simulink model "DP_STD_MDL_DCAC_3ph_2level_resload_2022b"  (R2022b)
settings: Solver=VariableStepAuto  StartTime=0.0  StopTime=6  RelTol=1e-3
libraries: spsSeriesRLCBranchLib x18, spsSecondOrderFilterLib x7, spsVoltageMeasurementLib x7, spsMosfetLib x4, simulink x2, spsControlledVoltageSourceLib x1, gmp_sil_core_pack x1, gmp_peripheral_utilities x1, spspowerguiLib x1
(part 1 of 2)
settings Model: SimulationMode=accelerator  Creator=javnson  LastModifiedBy=javnson
settings DataIOCC: ReturnWorkspaceOutputs=off
settings OptimizationCC: ReuseModelBlockBuffer=on
settings RTWCC: GPUComputeCapability=5.0

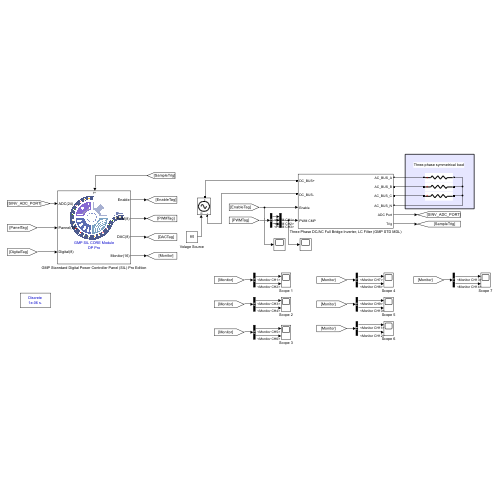
[thumbnail: Simulink's stored preview of the top-level diagram]
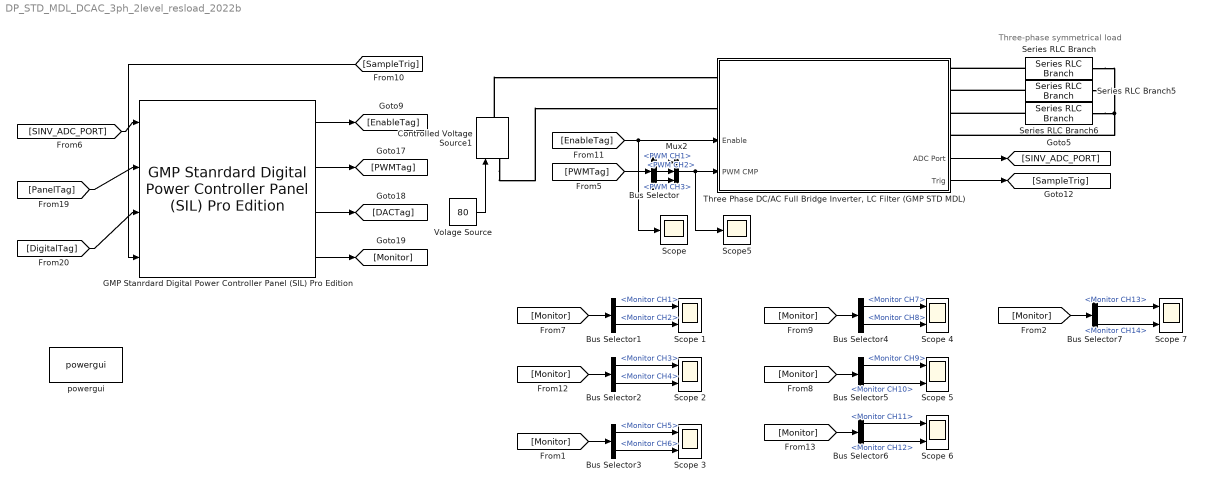
== system DP_STD_MDL_DCAC_3ph_2level_resload_2022b ==
  note: Three-phase symmetrical load
  Bus Selector : BusSelector  OutputSignals=PWM CH1,PWM CH2,PWM CH3
  Bus Selector1 : BusSelector  OutputSignals=Monitor CH1,Monitor CH2
  Bus Selector2 : BusSelector  OutputSignals=Monitor CH3,Monitor CH4
  Bus Selector3 : BusSelector  OutputSignals=Monitor CH5,Monitor CH6
  Bus Selector4 : BusSelector  OutputSignals=Monitor CH7,Monitor CH8
  Bus Selector5 : BusSelector  OutputSignals=Monitor CH9,Monitor CH10
  Bus Selector6 : BusSelector  OutputSignals=Monitor CH11,Monitor CH12
  Bus Selector7 : BusSelector  OutputSignals=Monitor CH13,Monitor CH14
  Controlled Voltage Source1 : spsControlledVoltageSourceLib/Controlled Voltage Source  Initialize=on  Source_Type=AC  Amplitude=0  Phase=0  Frequency=0  Measurements=None
  GMP Stanrdard Digital Power Controller Panel (SIL) Pro Edition : gmp_sil_core_pack/GMP Stanrdard Digital Power Controller Panel (SIL) Pro Edition
      settings: SourceProductName=GMP SIL Core Utilities
  Mux2 : Mux  Inputs=3
  Scope : Scope
  Scope {1..7} (7 alike) : Scope  NumInputPorts=2
  Scope5 : Scope
  Series RLC Branch : spsSeriesRLCBranchLib/Series RLC Branch  LConnTagsString=__new0  RConnTagsString=__new0  BranchType=R  Resistance=50/3  Inductance=1e-3  SetiL0=off  InitialCurrent=0  Capacitance=1e-6  Setx0=off  InitialVoltage=0  Measurements=None
  Series RLC Branch5 : spsSeriesRLCBranchLib/Series RLC Branch  LConnTagsString=__new0  RConnTagsString=__new0  BranchType=R  Resistance=50/3  Inductance=1e-3  SetiL0=off  InitialCurrent=0  Capacitance=1e-6  Setx0=off  InitialVoltage=0  Measurements=None
  Series RLC Branch6 : spsSeriesRLCBranchLib/Series RLC Branch  LConnTagsString=__new0  RConnTagsString=__new0  BranchType=R  Resistance=50/3  Inductance=1e-3  SetiL0=off  InitialCurrent=0  Capacitance=1e-6  Setx0=off  InitialVoltage=0  Measurements=None
  "Three Phase DC/AC Full Bridge Inverter, LC Filter (GMP STD MDL)" : Subsystem  mask{R_mosfet_on=0.001, Lon=0, Rd=0.01, Vf=0.5, Rs=1e5, Cs=inf, ACF_L=1.5e-3, ACF_L_ESR=50e-3, ACF_C=5e-6, ACF_C_ESR=0.09, ACF_C_EPR=10e3, DC_CAP=220e-6*3, DC_CAP_ESR=0.05, DC_CAP_EPR=10e3, fswitch=20e3, CMP_MAX=3000, Deadband_Upper=50, Deadband_Lower=50, phase_shift=0, ADC_Resolution=12, DC_Voltage_Gain=0.02738589, DC_VOLTAGE_ADC_REFERENCE=3.3, DC_VOLTAGE_ADC_BIAS=0, DC_VOLTAGE_ADC_CUT_FREQ=1e3, DC_BUS_CURRENT_SENSOR_R=0.001, DC_Current_Gain=24.75, DC_CURRENT_ADC_REFERENCE=3.3, DC_CURRENT_ADC_BIAS=1.65, DC_CURRENT_ADC_CUT_FREQ=100e3, AC_Voltage_Gain=0.04125, AC_VOLTAGE_ADC_REFERENCE=3.3, AC_VOLTAGE_ADC_BIAS=1.65, AC_VOLTAGE_ADC_CUT_FREQ=1e3, ADC_AC_R_SENSOR=0.001, AC_Current_Gain=48, AC_CURRENT_ADC_REFERENCE=3.3, AC_CURRENT_ADC_BIAS=1.65, AC_CURRENT_ADC_INIT=0, CAP_CURRENT_SENSOR_R=0.001, CAP_Current_Gain=20, CAP_CURRENT_ADC_REFERENCE=3.3, CAP_CURRENT_ADC_BIAS=1.65, CAP_CURRENT_ADC_CUT_FREQ=18e3, GRID_CURRENT_SENSOR_R=0.001, Grid_Current_Gain=48, GRID_CURRENT_ADC_REFERENCE=3.3, GRID_CURRENT_ADC_BIAS=1.65, GRID_CURRENT_ADC_CUT_FREQ=100e3}
      mask prompts: ADC_Resolution "ADC_BIT:"; DC_Voltage_Gain "ADC_GAIN:"; DC_VOLTAGE_ADC_REFERENCE "ADC_REFERENCE:"; DC_VOLTAGE_ADC_BIAS "ADC_BIAS:"; DC_VOLTAGE_ADC_CUT_FREQ "cut_frequency:"; DC_Current_Gain "ADC_GAIN:"; DC_CURRENT_ADC_REFERENCE "ADC_REFERENCE:"; DC_CURRENT_ADC_BIAS "ADC_BIAS:"; DC_CURRENT_ADC_CUT_FREQ "ADC_FILTER:"; AC_Voltage_Gain "ADC_GAIN:"; AC_VOLTAGE_ADC_REFERENCE "ADC_REFERENCE:"; AC_VOLTAGE_ADC_BIAS "ADC_BIAS:"; AC_VOLTAGE_ADC_CUT_FREQ "cut_frequency:"; ADC_AC_R_SENSOR "ADC_DC_R_SENSOR:"; AC_Current_Gain "ADC_GAIN:"; AC_CURRENT_ADC_REFERENCE "ADC_REFERENCE:"; AC_CURRENT_ADC_BIAS "ADC_BIAS:"; AC_CURRENT_ADC_INIT "ADC_INIT:"; CAP_CURRENT_SENSOR_R "CAP_BUS_CURRENT_SENSOR_R:"; CAP_Current_Gain "ADC_GAIN:"; CAP_CURRENT_ADC_REFERENCE "ADC_REFERENCE:"; CAP_CURRENT_ADC_BIAS "ADC_BIAS:"; CAP_CURRENT_ADC_CUT_FREQ "ADC_FILTER:"; GRID_CURRENT_SENSOR_R "DC_BUS_CURRENT_SENSOR_R:"; Grid_Current_Gain "ADC_GAIN:"; GRID_CURRENT_ADC_REFERENCE "ADC_REFERENCE:"; GRID_CURRENT_ADC_BIAS "ADC_BIAS:"; GRID_CURRENT_ADC_CUT_FREQ "ADC_FILTER:"
      settings: PortSchema="{\"entries\":[{\"content\":{\"sides\":[{\"content\":{\"connectorIds\":[\"LConn1\",\"LConn2\",\"In1\",\"In2\"]},\"type\":\"ConnectorPlacement.EquallySpacedRectSide\",\"uuid\":\"0e3e6e75-5e1a-455b-8a22-c69d0a4261ca\"},{\"content\":{\"connectorIds\":[\"RConn1\",\"RConn2\",\"RConn3\",\"RConn4\",\"Out1\",\"Out2\"],\"side\":\"RIGHT\"},\"type\":\"ConnectorPlacement.EquallySpacedRectSide\",\"uuid\":\"20326781-9238-4fea-80fd-ba96906d5d3f\"},{\"content\":{\"side\":\"TOP\"},\"type\":\"ConnectorPlacement.EquallySpacedRectSide\",\"uuid\":\"9e3289d3-0bee-4337-807b-c293a46cda9c\"}]},\"type\":\"ConnectorPlacement.EquallySpacedConnector\",\"uuid\":\"56bb35ad-d602-4874-b9bf-b95a81ef662c\"}],\"packageUris\":[\"http://schema.mathworks.com/mf0/Connector/R2020b\"],\"version\":\"1.0\"}"
      mask DialogControl ParameterGroupVar Prompt: 参数
      mask DialogControl Container4 Prompt: Component Parameters
      mask DialogControl Container7 Prompt: MOSFET
      mask DialogControl Control2 Prompt: Rds(on), unit Ohm
      mask DialogControl Control3 Prompt: Internal diode inducctance, unit H
      mask DialogControl Control4 Prompt: Internal diode resistance Rd, unit Ohm
      mask DialogControl Control5 Prompt: Internal diode forward voltage Vf, unit V
      mask DialogControl Control6 Prompt: Snubber resistance Rs, unit ohm
      mask DialogControl Control7 Prompt: Snubber Capacitance Cs, unit F
      mask DialogControl Container8 Prompt: LC Filter
      mask DialogControl Container20 Prompt: Filter Inductor
      mask DialogControl Control8 Prompt: AC Bus Filter Inductor (H)
      mask DialogControl Control42 Prompt: AC Bus Filter Inductor, ESR (Ohm)
      mask DialogControl Container21 Prompt: Filter Capcitor
      mask DialogControl Control43 Prompt: AC Bus Filter Capacitor (F)
      mask DialogControl Control44 Prompt: AC Bus Filter Capacitor, ESR (Ohm)
      mask DialogControl Control45 Prompt: AC Bus Filter Capacitor, EPR (Ohm)
      mask DialogControl Container22 Prompt: DC Bus Capacitor
      mask DialogControl Control46 Prompt: DC Bus Capacitor (F)
      mask DialogControl Control47 Prompt: DC Bus Capacitor, ESR (Ohm)
      mask DialogControl Control48 Prompt: DC Bus Capacitor, EPR (Ohm)
      mask DialogControl Container5 Prompt: PWM Parameers
      mask DialogControl Control9 Prompt: PWM Frequency (Hz):
      mask DialogControl Control10 Prompt: Full Scale PWM Compare value:
      mask DialogControl Control11 Prompt: (whole period is 2 * CMP_MAX ticks)
      mask DialogControl Control12 Prompt: Deadband Range Set (CMP Value):
      mask DialogControl Control13 Prompt: Single side deadband time: DEADBAND_CMP/2/CMP_MAX/fswitch
      mask DialogControl Control14 Prompt: Initial Phase Shift, unit rad
      mask DialogControl Container6 Prompt: ADC Parameters
      mask DialogControl Container14 Prompt: ADC Device
      mask DialogControl Control15 Prompt: ADC resolution:
      mask DialogControl Container15 Prompt: DC Side Voltage Sensor
      mask DialogControl Control16 Prompt: ADC Voltage Gain (Scale Factor):
      mask DialogControl Control17 Prompt: ADC reference Voltage(V)
      mask DialogControl Control18 Prompt: ADC Bias Voltage(V)
      mask DialogControl Control19 Prompt: Voltage Filter cut frequency (Hz):
      mask DialogControl Control20 Prompt: Generally, this value less than switch frequency / 10, greater than motor normal frequency * 3
      mask DialogControl Container16 Prompt: DC Side Current Sensor
      mask DialogControl Control26 Prompt: DC Bus Current Sensor Resistance
      mask DialogControl Control34 Prompt: ADC Current Gain (Scale Factor):
      mask DialogControl Control27 Prompt: ADC reference Voltage(V), ADC full scale current (when gain = 1)
      mask DialogControl Control28 Prompt: ADC Bias Current(A)
      mask DialogControl Control35 Prompt: Voltage Filter cut frequency (Hz):
      mask DialogControl Control36 Prompt: Generally, this value less than switch frequency / 10, greater than motor normal frequency * 3
      mask DialogControl Container17 Prompt: AC Side Voltage Sensor
      mask DialogControl Control16_copy Prompt: ADC Voltage Gain (Scale Factor):
      mask DialogControl Control17_copy Prompt: ADC reference Voltage(V)
      mask DialogControl Control18_copy Prompt: ADC Bias Voltage(V)
      mask DialogControl Control19_copy Prompt: Voltage Filter cut frequency (Hz):
      mask DialogControl Control20_copy Prompt: Generally, this value less than switch frequency / 10, greater than motor normal frequency * 3
      mask DialogControl Container18 Prompt: AC Side Current Sensor(NC)
      mask DialogControl Control55 Prompt: AC Current Sensor Resistance
      mask DialogControl Control26_copy Prompt: ADC Current Gain (Scale Factor):
      mask DialogControl Control27_copy Prompt: ADC reference Current(A), ADC full scale current (when gain = 1)
      mask DialogControl Control28_copy Prompt: ADC Bias Current(A)
      mask DialogControl Control29_copy Prompt: ADC initial Current Output(A)
      mask DialogControl Container19 Prompt: Capcitor Current Sensor(NC)
      mask DialogControl Control26_copy_copy Prompt: Filter Capacitor Current Sensor Resistance
      mask DialogControl Control34_copy Prompt: ADC Current Gain (Scale Factor):
      mask DialogControl Control27_copy_copy Prompt: ADC reference Voltage(V), ADC full scale current (when gain = 1)
      mask DialogControl Control28_copy_copy Prompt: ADC Bias Current(V)
      mask DialogControl Control35_copy Prompt: Voltage Filter cut frequency (Hz):
      mask DialogControl Control36_copy Prompt: Generally, this value less than switch frequency / 10, greater than motor normal frequency * 3
      mask DialogControl Container23 Prompt: Grid Current Sensor
      mask DialogControl Control26_copy_copy_copy Prompt: Grid Bus Current Sensor Resistance
      mask DialogControl Control34_copy_copy Prompt: ADC Current Gain (Scale Factor):
      mask DialogControl Control27_copy_copy_copy Prompt: ADC reference Voltage(V), ADC full scale current (when gain = 1)
      mask DialogControl Control28_copy_copy_copy Prompt: ADC Bias Current(V)
      mask DialogControl Control35_copy_copy Prompt: Voltage Filter cut frequency (Hz):
      mask DialogControl Control36_copy_copy Prompt: Generally, this value less than switch frequency / 10, greater than motor normal frequency * 3
  Volage Source : Constant  Value=80
  powergui : spspowerguiLib/powergui  Priority=1  SimulationMode=Discrete  SampleTime=1e-6  frequency=60  Iterations=50  frequencyindice=0  Pbase=100e6  ErrMax=1e-4  UnitsV=kV  UnitsW=MW  buscounter=0  FunctionMessages=off  echomessages=off  EnableUseOfTLC=off  CurrentSourceSwitches=off  DisableSnubberDevices=off  DisableRonSwitches=off  DisableVfSwitches=off  DisplayEquations=off  AutomaticDiscreteSolvers=off  SolverType=Tustin/Backward Euler (TBE)  Interpol=off  ExternalGateDelay=off  methode=off  Ts=100  x0status=blocks  SPID=on  SwTol=0  HookPort=off  NonlinearTolerance=1e-4  nMaxIteration=100  ContinueOnMaxIteration=off  RestoreLinks=warning  ResistiveCurrentMeasurement=off  Frange=[0:2:500]  Ylog=off  Xlog=on  ShowGrid=off  save=off  variable=ZData  structure=0  ZoomFFT=off  StartTime=0.0  cycles=1  DisplayStyle=1  fundamental=60  FreqAxis=off  MaxFrequency=1000  frequencyindicesteady=1  RmsSteady=1  display=off
  wires:
  Volage Source/1 -> Controlled Voltage Source1/1
  [EnableTag] -> "Three Phase DC/AC Full Bridge Inverter, LC Filter (GMP STD MDL)"/1(Enable), Scope/1
  [SampleTrig] -> GMP Stanrdard Digital Power Controller Panel (SIL) Pro Edition/4
  GMP Stanrdard Digital Power Controller Panel (SIL) Pro Edition/1 -> [EnableTag]
  GMP Stanrdard Digital Power Controller Panel (SIL) Pro Edition/2 -> [PWMTag]
  GMP Stanrdard Digital Power Controller Panel (SIL) Pro Edition/3 -> [DACTag]
  GMP Stanrdard Digital Power Controller Panel (SIL) Pro Edition/4 -> [Monitor]
  [SINV_ADC_PORT] -> GMP Stanrdard Digital Power Controller Panel (SIL) Pro Edition/1
  [PanelTag] -> GMP Stanrdard Digital Power Controller Panel (SIL) Pro Edition/2
  [DigitalTag] -> GMP Stanrdard Digital Power Controller Panel (SIL) Pro Edition/3
  [PWMTag] -> Bus Selector/1
  Bus Selector/1 -> Mux2/1  "<PWM CH1>"
  Bus Selector/2 -> Mux2/2  "<PWM CH2>"
  Mux2/1 -> "Three Phase DC/AC Full Bridge Inverter, LC Filter (GMP STD MDL)"/2(PWM CMP), Scope5/1
  [Monitor] -> Bus Selector1/1
  Bus Selector1/1 -> Scope 1/1  "<Monitor CH1>"
  Bus Selector1/2 -> Scope 1/2  "<Monitor CH2>"
  [Monitor] -> Bus Selector2/1
  Bus Selector2/1 -> Scope 2/1  "<Monitor CH3>"
  Bus Selector2/2 -> Scope 2/2  "<Monitor CH4>"
  Bus Selector3/2 -> Scope 3/2  "<Monitor CH6>"
  Bus Selector3/1 -> Scope 3/1  "<Monitor CH5>"
  [Monitor] -> Bus Selector3/1
  Bus Selector5/2 -> Scope 5/2  "<Monitor CH10>"
  Bus Selector5/1 -> Scope 5/1  "<Monitor CH9>"
  [Monitor] -> Bus Selector5/1
  [Monitor] -> Bus Selector4/1
  Bus Selector4/1 -> Scope 4/1  "<Monitor CH7>"
  Bus Selector4/2 -> Scope 4/2  "<Monitor CH8>"
  [Monitor] -> Bus Selector6/1
  Bus Selector6/1 -> Scope 6/1  "<Monitor CH11>"
  "Three Phase DC/AC Full Bridge Inverter, LC Filter (GMP STD MDL)"/1(ADC Port) -> [SINV_ADC_PORT]
  "Three Phase DC/AC Full Bridge Inverter, LC Filter (GMP STD MDL)"/2(Trig) -> [SampleTrig]
  Bus Selector/3 -> Mux2/3  "<PWM CH3>"
  Bus Selector6/2 -> Scope 6/2  "<Monitor CH12>"
  Bus Selector7/2 -> Scope 7/2  "<Monitor CH14>"
  Bus Selector7/1 -> Scope 7/1  "<Monitor CH13>"
  [Monitor] -> Bus Selector7/1
  connections:
  Controlled Voltage Source1/LConn1 -- "Three Phase DC/AC Full Bridge Inverter, LC Filter (GMP STD MDL)"/LConn2
  Controlled Voltage Source1/RConn1 -- "Three Phase DC/AC Full Bridge Inverter, LC Filter (GMP STD MDL)"/LConn1
  Series RLC Branch/LConn1 -- "Three Phase DC/AC Full Bridge Inverter, LC Filter (GMP STD MDL)"/RConn1
  Series RLC Branch5/LConn1 -- "Three Phase DC/AC Full Bridge Inverter, LC Filter (GMP STD MDL)"/RConn2
  Series RLC Branch6/LConn1 -- "Three Phase DC/AC Full Bridge Inverter, LC Filter (GMP STD MDL)"/RConn3
  Series RLC Branch/RConn1 -- Series RLC Branch5/RConn1 -- Series RLC Branch6/RConn1 -- "Three Phase DC/AC Full Bridge Inverter, LC Filter (GMP STD MDL)"/RConn4

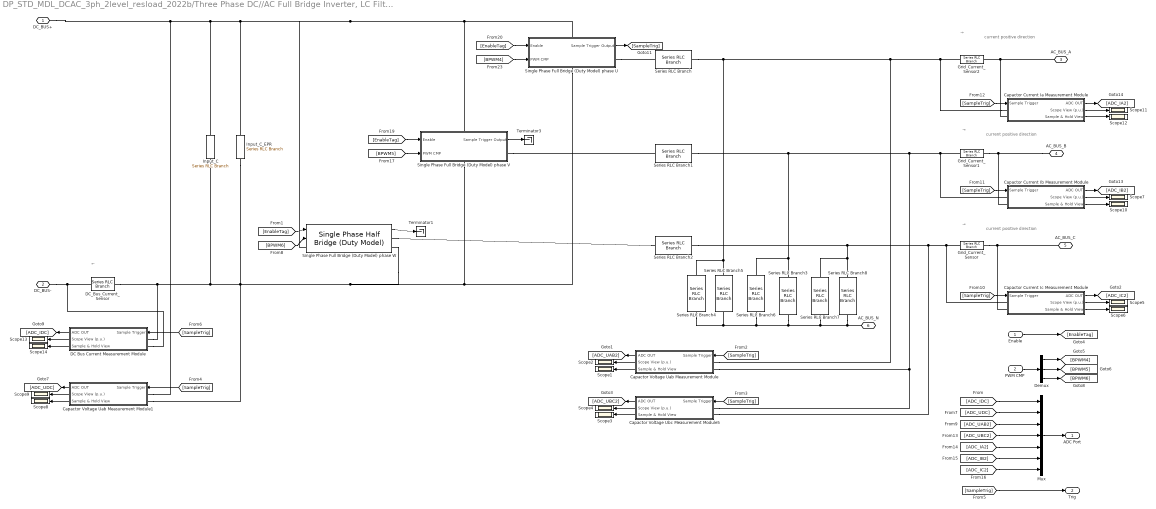
== system DP_STD_MDL_DCAC_3ph_2level_resload_2022b/Three Phase DC//AC Full Bridge Inverter, LC Filter (GMP STD MDL) ==
  note: ←
  note: →
  note: current positive direction
  note: →
  note: current positive direction
  note: →
  note: current positive direction
  Enable : Inport
  PWM CMP : Inport  Port=2
  Capactor Current Ia Measurement Module : Subsystem  mask{ADC_GAIN=Grid_Current_Gain, ADC_BIT=ADC_Resolution, ADC_REFERENCE=GRID_CURRENT_ADC_REFERENCE, ADC_BIAS=GRID_CURRENT_ADC_BIAS, ADC_INIT=0, cut_frequency=GRID_CURRENT_ADC_CUT_FREQ}
      mask DialogControl DescGroupVar Prompt: Voltage Sample ADC Model
      mask DialogControl DescTextVar Prompt: This is a ideal Voltage Measurement Module.
      mask DialogControl Control2 Prompt: ADC(p.u.) = (real_voltage * ADC_GAIN + ADC_BIAS)/ADC_REFERENCE
      mask DialogControl Control11 Prompt: GMP CTL Simulink Utilities: virtual peripherals
      mask DialogControl ParameterGroupVar Prompt: Parameters:
      mask DialogControl Control4 Prompt: ADC Voltage Gain (Scale Factor):
      mask DialogControl Control5 Prompt: ADC resolution:
      mask DialogControl Control6 Prompt: ADC reference Voltage(V)
      mask DialogControl Control8 Prompt: ADC Bias Voltage(V)
      mask DialogControl Control7 Prompt: ADC Initial Voltage Output (V):
      mask DialogControl Control9 Prompt: Voltage Filter cut frequency (Hz):
      mask DialogControl Control10 Prompt: Generally, this value less than switch frequency / 10, greater than motor normal frequency * 3
  Capactor Current Ib Measurement Module : Subsystem  mask{ADC_GAIN=Grid_Current_Gain, ADC_BIT=ADC_Resolution, ADC_REFERENCE=GRID_CURRENT_ADC_REFERENCE, ADC_BIAS=GRID_CURRENT_ADC_BIAS, ADC_INIT=0, cut_frequency=GRID_CURRENT_ADC_CUT_FREQ}
      mask DialogControl DescGroupVar Prompt: Voltage Sample ADC Model
      mask DialogControl DescTextVar Prompt: This is a ideal Voltage Measurement Module.
      mask DialogControl Control2 Prompt: ADC(p.u.) = (real_voltage * ADC_GAIN + ADC_BIAS)/ADC_REFERENCE
      mask DialogControl Control11 Prompt: GMP CTL Simulink Utilities: virtual peripherals
      mask DialogControl ParameterGroupVar Prompt: Parameters:
      mask DialogControl Control4 Prompt: ADC Voltage Gain (Scale Factor):
      mask DialogControl Control5 Prompt: ADC resolution:
      mask DialogControl Control6 Prompt: ADC reference Voltage(V)
      mask DialogControl Control8 Prompt: ADC Bias Voltage(V)
      mask DialogControl Control7 Prompt: ADC Initial Voltage Output (V):
      mask DialogControl Control9 Prompt: Voltage Filter cut frequency (Hz):
      mask DialogControl Control10 Prompt: Generally, this value less than switch frequency / 10, greater than motor normal frequency * 3
  Capactor Current Ic Measurement Module : Subsystem  mask{ADC_GAIN=Grid_Current_Gain, ADC_BIT=ADC_Resolution, ADC_REFERENCE=GRID_CURRENT_ADC_REFERENCE, ADC_BIAS=GRID_CURRENT_ADC_BIAS, ADC_INIT=0, cut_frequency=GRID_CURRENT_ADC_CUT_FREQ}
      mask DialogControl DescGroupVar Prompt: Voltage Sample ADC Model
      mask DialogControl DescTextVar Prompt: This is a ideal Voltage Measurement Module.
      mask DialogControl Control2 Prompt: ADC(p.u.) = (real_voltage * ADC_GAIN + ADC_BIAS)/ADC_REFERENCE
      mask DialogControl Control11 Prompt: GMP CTL Simulink Utilities: virtual peripherals
      mask DialogControl ParameterGroupVar Prompt: Parameters:
      mask DialogControl Control4 Prompt: ADC Voltage Gain (Scale Factor):
      mask DialogControl Control5 Prompt: ADC resolution:
      mask DialogControl Control6 Prompt: ADC reference Voltage(V)
      mask DialogControl Control8 Prompt: ADC Bias Voltage(V)
      mask DialogControl Control7 Prompt: ADC Initial Voltage Output (V):
      mask DialogControl Control9 Prompt: Voltage Filter cut frequency (Hz):
      mask DialogControl Control10 Prompt: Generally, this value less than switch frequency / 10, greater than motor normal frequency * 3
  Capactor Voltage Uab Measurement Module : Subsystem  mask{ADC_GAIN=AC_Voltage_Gain, ADC_BIT=ADC_Resolution, ADC_REFERENCE=AC_VOLTAGE_ADC_REFERENCE, ADC_BIAS=AC_VOLTAGE_ADC_BIAS, ADC_INIT=0, cut_frequency=AC_VOLTAGE_ADC_CUT_FREQ}
      mask DialogControl DescGroupVar Prompt: Voltage Sample ADC Model
      mask DialogControl DescTextVar Prompt: This is a ideal Voltage Measurement Module.
      mask DialogControl Control2 Prompt: ADC(p.u.) = (real_voltage * ADC_GAIN + ADC_BIAS)/ADC_REFERENCE
      mask DialogControl Control11 Prompt: GMP CTL Simulink Utilities: virtual peripherals
      mask DialogControl ParameterGroupVar Prompt: Parameters:
      mask DialogControl Control4 Prompt: ADC Voltage Gain (Scale Factor):
      mask DialogControl Control5 Prompt: ADC resolution:
      mask DialogControl Control6 Prompt: ADC reference Voltage(V)
      mask DialogControl Control8 Prompt: ADC Bias Voltage(V)
      mask DialogControl Control7 Prompt: ADC Initial Voltage Output (V):
      mask DialogControl Control9 Prompt: Voltage Filter cut frequency (Hz):
      mask DialogControl Control10 Prompt: Generally, this value less than switch frequency / 10, greater than motor normal frequency * 3
  Capactor Voltage Uab Measurement Module1 : Subsystem  mask{ADC_GAIN=DC_Voltage_Gain, ADC_BIT=ADC_Resolution, ADC_REFERENCE=DC_VOLTAGE_ADC_REFERENCE, ADC_BIAS=DC_VOLTAGE_ADC_BIAS, ADC_INIT=0, cut_frequency=DC_VOLTAGE_ADC_CUT_FREQ}
      mask DialogControl DescGroupVar Prompt: Voltage Sample ADC Model
      mask DialogControl DescTextVar Prompt: This is a ideal Voltage Measurement Module.
      mask DialogControl Control2 Prompt: ADC(p.u.) = (real_voltage * ADC_GAIN + ADC_BIAS)/ADC_REFERENCE
      mask DialogControl Control11 Prompt: GMP CTL Simulink Utilities: virtual peripherals
      mask DialogControl ParameterGroupVar Prompt: Parameters:
      mask DialogControl Control4 Prompt: ADC Voltage Gain (Scale Factor):
      mask DialogControl Control5 Prompt: ADC resolution:
      mask DialogControl Control6 Prompt: ADC reference Voltage(V)
      mask DialogControl Control8 Prompt: ADC Bias Voltage(V)
      mask DialogControl Control7 Prompt: ADC Initial Voltage Output (V):
      mask DialogControl Control9 Prompt: Voltage Filter cut frequency (Hz):
      mask DialogControl Control10 Prompt: Generally, this value less than switch frequency / 10, greater than motor normal frequency * 3
  Capactor Voltage Ubc Measurement Module5 : Subsystem  mask{ADC_GAIN=AC_Voltage_Gain, ADC_BIT=ADC_Resolution, ADC_REFERENCE=AC_VOLTAGE_ADC_REFERENCE, ADC_BIAS=AC_VOLTAGE_ADC_BIAS, ADC_INIT=0, cut_frequency=AC_VOLTAGE_ADC_CUT_FREQ}
      mask DialogControl DescGroupVar Prompt: Voltage Sample ADC Model
      mask DialogControl DescTextVar Prompt: This is a ideal Voltage Measurement Module.
      mask DialogControl Control2 Prompt: ADC(p.u.) = (real_voltage * ADC_GAIN + ADC_BIAS)/ADC_REFERENCE
      mask DialogControl Control11 Prompt: GMP CTL Simulink Utilities: virtual peripherals
      mask DialogControl ParameterGroupVar Prompt: Parameters:
      mask DialogControl Control4 Prompt: ADC Voltage Gain (Scale Factor):
      mask DialogControl Control5 Prompt: ADC resolution:
      mask DialogControl Control6 Prompt: ADC reference Voltage(V)
      mask DialogControl Control8 Prompt: ADC Bias Voltage(V)
      mask DialogControl Control7 Prompt: ADC Initial Voltage Output (V):
      mask DialogControl Control9 Prompt: Voltage Filter cut frequency (Hz):
      mask DialogControl Control10 Prompt: Generally, this value less than switch frequency / 10, greater than motor normal frequency * 3
  DC Bus Current Measurement Module : Subsystem  mask{ADC_GAIN=DC_Current_Gain, ADC_BIT=ADC_Resolution, ADC_REFERENCE=DC_CURRENT_ADC_REFERENCE, ADC_BIAS=DC_CURRENT_ADC_BIAS, ADC_INIT=0, cut_frequency=DC_CURRENT_ADC_CUT_FREQ}
      mask DialogControl DescGroupVar Prompt: Voltage Sample ADC Model
      mask DialogControl DescTextVar Prompt: This is a ideal Voltage Measurement Module.
      mask DialogControl Control2 Prompt: ADC(p.u.) = (real_voltage * ADC_GAIN + ADC_BIAS)/ADC_REFERENCE
      mask DialogControl Control11 Prompt: GMP CTL Simulink Utilities: virtual peripherals
      mask DialogControl ParameterGroupVar Prompt: Parameters:
      mask DialogControl Control4 Prompt: ADC Voltage Gain (Scale Factor):
      mask DialogControl Control5 Prompt: ADC resolution:
      mask DialogControl Control6 Prompt: ADC reference Voltage(V)
      mask DialogControl Control8 Prompt: ADC Bias Voltage(V)
      mask DialogControl Control7 Prompt: ADC Initial Voltage Output (V):
      mask DialogControl Control9 Prompt: Voltage Filter cut frequency (Hz):
      mask DialogControl Control10 Prompt: Generally, this value less than switch frequency / 10, greater than motor normal frequency * 3
  DC_Bus_Current_Sensor : spsSeriesRLCBranchLib/Series RLC Branch  LConnTagsString=__new0  RConnTagsString=__new0  BranchType=R  Resistance=DC_BUS_CURRENT_SENSOR_R  Inductance=695e-6  SetiL0=off  InitialCurrent=0  Capacitance=ACF_C  Setx0=off  InitialVoltage=0  Measurements=None
  Demux : Demux  Outputs=3
  Grid_Current_Sensor : spsSeriesRLCBranchLib/Series RLC Branch  LConnTagsString=__new0  RConnTagsString=__new0  BranchType=R  Resistance=GRID_CURRENT_SENSOR_R  Inductance=1e-3  SetiL0=off  InitialCurrent=0  Capacitance=1e-6  Setx0=off  InitialVoltage=0  Measurements=None
  Grid_Current_Sensor1 : spsSeriesRLCBranchLib/Series RLC Branch  LConnTagsString=__new0  RConnTagsString=__new0  BranchType=R  Resistance=GRID_CURRENT_SENSOR_R  Inductance=1e-3  SetiL0=off  InitialCurrent=0  Capacitance=1e-6  Setx0=off  InitialVoltage=0  Measurements=None
  Grid_Current_Sensor2 : spsSeriesRLCBranchLib/Series RLC Branch  LConnTagsString=__new0  RConnTagsString=__new0  BranchType=R  Resistance=GRID_CURRENT_SENSOR_R  Inductance=1e-3  SetiL0=off  InitialCurrent=0  Capacitance=1e-6  Setx0=off  InitialVoltage=0  Measurements=None
  Input_C : spsSeriesRLCBranchLib/Series RLC Branch  LConnTagsString=__new0  RConnTagsString=__new0  BranchType=RC  Resistance=DC_CAP_ESR  Inductance=1e-3  SetiL0=off  InitialCurrent=0  Capacitance=DC_CAP  Setx0=off  InitialVoltage=0  Measurements=None
  Input_C_EPR : spsSeriesRLCBranchLib/Series RLC Branch  LConnTagsString=__new0  RConnTagsString=__new0  BranchType=R  Resistance=DC_CAP_EPR  Inductance=1e-3  SetiL0=off  InitialCurrent=0  Capacitance=1e-6  Setx0=off  InitialVoltage=0  Measurements=None
  Mux : Mux  Inputs=7
  Scope{1..14} (14 alike) : Scope
  Series RLC Branch : spsSeriesRLCBranchLib/Series RLC Branch  LConnTagsString=__new0  RConnTagsString=__new0  BranchType=RL  Resistance=ACF_L_ESR  Inductance=ACF_L  SetiL0=off  InitialCurrent=0  Capacitance=1e-6  Setx0=off  InitialVoltage=0  Measurements=None
  Series RLC Branch1 : spsSeriesRLCBranchLib/Series RLC Branch  LConnTagsString=__new0  RConnTagsString=__new0  BranchType=RL  Resistance=ACF_L_ESR  Inductance=ACF_L  SetiL0=off  InitialCurrent=0  Capacitance=1e-6  Setx0=off  InitialVoltage=0  Measurements=None
  Series RLC Branch2 : spsSeriesRLCBranchLib/Series RLC Branch  LConnTagsString=__new0  RConnTagsString=__new0  BranchType=RL  Resistance=ACF_L_ESR  Inductance=ACF_L  SetiL0=off  InitialCurrent=0  Capacitance=1e-6  Setx0=off  InitialVoltage=0  Measurements=None
  Series RLC Branch3 : spsSeriesRLCBranchLib/Series RLC Branch  LConnTagsString=__new0  RConnTagsString=__new0  BranchType=RC  Resistance=ACF_C_ESR  Inductance=695e-6  SetiL0=off  InitialCurrent=0  Capacitance=ACF_C  Setx0=off  InitialVoltage=0  Measurements=None
  Series RLC Branch4 : spsSeriesRLCBranchLib/Series RLC Branch  LConnTagsString=__new0  RConnTagsString=__new0  BranchType=R  Resistance=DC_CAP_EPR  Inductance=695e-6  SetiL0=off  InitialCurrent=0  Capacitance=ACF_C  Setx0=off  InitialVoltage=0  Measurements=None
  Series RLC Branch5 : spsSeriesRLCBranchLib/Series RLC Branch  LConnTagsString=__new0  RConnTagsString=__new0  BranchType=RC  Resistance=ACF_C_ESR  Inductance=695e-6  SetiL0=off  InitialCurrent=0  Capacitance=ACF_C  Setx0=off  InitialVoltage=0  Measurements=None
  Series RLC Branch6 : spsSeriesRLCBranchLib/Series RLC Branch  LConnTagsString=__new0  RConnTagsString=__new0  BranchType=R  Resistance=DC_CAP_EPR  Inductance=695e-6  SetiL0=off  InitialCurrent=0  Capacitance=ACF_C  Setx0=off  InitialVoltage=0  Measurements=None
  Series RLC Branch7 : spsSeriesRLCBranchLib/Series RLC Branch  LConnTagsString=__new0  RConnTagsString=__new0  BranchType=R  Resistance=DC_CAP_EPR  Inductance=695e-6  SetiL0=off  InitialCurrent=0  Capacitance=ACF_C  Setx0=off  InitialVoltage=0  Measurements=None
  Series RLC Branch8 : spsSeriesRLCBranchLib/Series RLC Branch  LConnTagsString=__new0  RConnTagsString=__new0  BranchType=RC  Resistance=ACF_C_ESR  Inductance=695e-6  SetiL0=off  InitialCurrent=0  Capacitance=ACF_C  Setx0=off  InitialVoltage=0  Measurements=None
  Single Phase Full Bridge (Duty Model) phase U : Subsystem  mask{fswitch=fswitch, CMP_MAX=CMP_MAX, Deadband_Upper=Deadband_Upper, Deadband_Lower=Deadband_Lower, Deadband_us=NaN, phase_shift=0, R_mosfet_on=0.1, Lon=0, Rd=0.01, Vf=0.3, Rs=1e5, Cs=inf}
      mask init:
      | calculate_deadband(gcb, 'Deadband_Upper', 'Deadband_Lower',	'CMP_MAX', 'fswitch', 'Deadband_us');
      settings: PortSchema="{\"entries\":[{\"content\":{\"sides\":[{\"content\":{\"connectorIds\":[\"In1\",\"In2\"]},\"type\":\"ConnectorPlacement.EquallySpacedRectSide\",\"uuid\":\"20beeabc-b0ca-4337-b227-c7f02abd15d8\"},{\"content\":{\"connectorIds\":[\"Out1\",\"RConn1\"],\"side\":\"RIGHT\"},\"type\":\"ConnectorPlacement.EquallySpacedRectSide\",\"uuid\":\"a7923383-ac55-4621-ad1d-4d067c1fb84d\"},{\"content\":{\"connectorIds\":[\"LConn1\"],\"side\":\"TOP\"},\"type\":\"ConnectorPlacement.EquallySpacedRectSide\",\"uuid\":\"661bf0ae-1c96-4de8-96aa-28c06a0a56db\"},{\"content\":{\"connectorIds\":[\"RConn2\"],\"side\":\"BOTTOM\"},\"type\":\"ConnectorPlacement.EquallySpacedRectSide\",\"uuid\":\"fc2f6321-5787-4e1a-b5a2-65ed34db36b5\"}]},\"type\":\"ConnectorPlacement.EquallySpacedConnector\",\"uuid\":\"e2219b16-0a50-43ef-8183-c55a35d5a2a0\"}],\"packageUris\":[\"http://schema.mathworks.com/mf0/Connector/R2020b\"],\"version\":\"1.0\"}"
      mask Callback fswitch: calculate_deadband(gcb, 'Deadband_Upper', 'Deadband_Lower',	'CMP_MAX', 'fswitch', 'Deadband_us');
      mask Callback CMP_MAX: calculate_deadband(gcb, 'Deadband_Upper', 'Deadband_Lower',	'CMP_MAX', 'fswitch', 'Deadband_us');
      mask Callback Deadband_Upper: calculate_deadband(gcb, 'Deadband_Upper', 'Deadband_Lower',	'CMP_MAX', 'fswitch', 'Deadband_us');
      mask Callback Deadband_Lower: calculate_deadband(gcb, 'Deadband_Upper', 'Deadband_Lower',	'CMP_MAX', 'fswitch', 'Deadband_us');
      mask DialogControl DescGroupVar Prompt: Half Bridge With PWM Module
      mask DialogControl Control14 Prompt: GMP CTL Simulink Utilities: virtual peripherals
      mask DialogControl DescTextVar Prompt: This module provide a PWM (with deadband), and a MOSFET half bridge.
      mask DialogControl Container5 Prompt: PWM Modulator
      mask DialogControl ParameterGroupVar Prompt: PWM module parameters
      mask DialogControl Control2 Prompt: PWM Frequency (Hz):
      mask DialogControl Control3 Prompt: Full Scale PWM Compare value:
      mask DialogControl Control4 Prompt: (whole period is 2 * CMP_MAX ticks)
      mask DialogControl Control5 Prompt: Deadband Range Set (CMP Value):
      mask DialogControl Control6 Prompt: Single side deadband time: DEADBAND_CMP/2/CMP_MAX/fswitch
      mask DialogControl Control15 Prompt: Calculated Deadband, us
      mask DialogControl Control13 Prompt: Initial Phase Shift, unit rad
      mask DialogControl Container6 Prompt: MOSFET
      mask DialogControl Container3 Prompt: MOSFET parameters
      mask DialogControl Control7 Prompt: Rds(on), unit Ohm
      mask DialogControl Control8 Prompt: Internal diode inducctance, unit H
      mask DialogControl Control9 Prompt: Internal diode resistance Rd, unit Ohm
      mask DialogControl Control10 Prompt: Internal diode forward voltage Vf, unit V
      mask DialogControl Control11 Prompt: Snubber resistance Rs, unit ohm
      mask DialogControl Control12 Prompt: Snubber Capacitance Cs, unit F
  Single Phase Full Bridge (Duty Model) phase V : Subsystem  mask{fswitch=fswitch, CMP_MAX=CMP_MAX, Deadband_Upper=Deadband_Upper, Deadband_Lower=Deadband_Lower, Deadband_us=NaN, phase_shift=0, R_mosfet_on=0.1, Lon=0, Rd=0.01, Vf=0.3, Rs=1e5, Cs=inf}
      mask init:
      | calculate_deadband(gcb, 'Deadband_Upper', 'Deadband_Lower',	'CMP_MAX', 'fswitch', 'Deadband_us');
      settings: PortSchema="{\"entries\":[{\"content\":{\"sides\":[{\"content\":{\"connectorIds\":[\"In1\",\"In2\"]},\"type\":\"ConnectorPlacement.EquallySpacedRectSide\",\"uuid\":\"20beeabc-b0ca-4337-b227-c7f02abd15d8\"},{\"content\":{\"connectorIds\":[\"Out1\",\"RConn1\"],\"side\":\"RIGHT\"},\"type\":\"ConnectorPlacement.EquallySpacedRectSide\",\"uuid\":\"a7923383-ac55-4621-ad1d-4d067c1fb84d\"},{\"content\":{\"connectorIds\":[\"LConn1\"],\"side\":\"TOP\"},\"type\":\"ConnectorPlacement.EquallySpacedRectSide\",\"uuid\":\"661bf0ae-1c96-4de8-96aa-28c06a0a56db\"},{\"content\":{\"connectorIds\":[\"RConn2\"],\"side\":\"BOTTOM\"},\"type\":\"ConnectorPlacement.EquallySpacedRectSide\",\"uuid\":\"fc2f6321-5787-4e1a-b5a2-65ed34db36b5\"}]},\"type\":\"ConnectorPlacement.EquallySpacedConnector\",\"uuid\":\"e2219b16-0a50-43ef-8183-c55a35d5a2a0\"}],\"packageUris\":[\"http://schema.mathworks.com/mf0/Connector/R2020b\"],\"version\":\"1.0\"}"
      mask Callback fswitch: calculate_deadband(gcb, 'Deadband_Upper', 'Deadband_Lower',	'CMP_MAX', 'fswitch', 'Deadband_us');
      mask Callback CMP_MAX: calculate_deadband(gcb, 'Deadband_Upper', 'Deadband_Lower',	'CMP_MAX', 'fswitch', 'Deadband_us');
      mask Callback Deadband_Upper: calculate_deadband(gcb, 'Deadband_Upper', 'Deadband_Lower',	'CMP_MAX', 'fswitch', 'Deadband_us');
      mask Callback Deadband_Lower: calculate_deadband(gcb, 'Deadband_Upper', 'Deadband_Lower',	'CMP_MAX', 'fswitch', 'Deadband_us');
      mask DialogControl DescGroupVar Prompt: Half Bridge With PWM Module
      mask DialogControl Control14 Prompt: GMP CTL Simulink Utilities: virtual peripherals
      mask DialogControl DescTextVar Prompt: This module provide a PWM (with deadband), and a MOSFET half bridge.
      mask DialogControl Container5 Prompt: PWM Modulator
      mask DialogControl ParameterGroupVar Prompt: PWM module parameters
      mask DialogControl Control2 Prompt: PWM Frequency (Hz):
      mask DialogControl Control3 Prompt: Full Scale PWM Compare value:
      mask DialogControl Control4 Prompt: (whole period is 2 * CMP_MAX ticks)
      mask DialogControl Control5 Prompt: Deadband Range Set (CMP Value):
      mask DialogControl Control6 Prompt: Single side deadband time: DEADBAND_CMP/2/CMP_MAX/fswitch
      mask DialogControl Control15 Prompt: Calculated Deadband, us
      mask DialogControl Control13 Prompt: Initial Phase Shift, unit rad
      mask DialogControl Container6 Prompt: MOSFET
      mask DialogControl Container3 Prompt: MOSFET parameters
      mask DialogControl Control7 Prompt: Rds(on), unit Ohm
      mask DialogControl Control8 Prompt: Internal diode inducctance, unit H
      mask DialogControl Control9 Prompt: Internal diode resistance Rd, unit Ohm
      mask DialogControl Control10 Prompt: Internal diode forward voltage Vf, unit V
      mask DialogControl Control11 Prompt: Snubber resistance Rs, unit ohm
      mask DialogControl Control12 Prompt: Snubber Capacitance Cs, unit F
  Single Phase Full Bridge (Duty Model) phase W : gmp_peripheral_utilities/Single Phase Half Bridge (Duty Model)  fswitch=fswitch  CMP_MAX=CMP_MAX  Deadband_Upper=Deadband_Upper  Deadband_Lower=Deadband_Lower  Deadband_us=NaN  phase_shift=0  R_mosfet_on=0.1  Lon=0  Rd=0.01  Vf=0.3  Rs=1e5  Cs=inf
      settings: SourceProductName=Virtual Peripheral Utilities
  Terminator1 : Terminator
  Terminator3 : Terminator
  DC_BUS+ : PMIOPort  Side=Left
  DC_BUS- : PMIOPort  Port=2  Side=Left
  AC_BUS_A : PMIOPort  Port=3  Side=Right
  AC_BUS_B : PMIOPort  Port=4  Side=Right
  AC_BUS_C : PMIOPort  Port=5  Side=Right
  AC_BUS_N : PMIOPort  Port=6  Side=Right
  ADC Port : Outport
  Trig : Outport  Port=2
  wires:
  [ADC_IC2] -> Mux/7
  [ADC_IB2] -> Mux/6
  [ADC_IA2] -> Mux/5
  [ADC_UBC2] -> Mux/4
  [ADC_UAB2] -> Mux/3
  [ADC_UDC] -> Mux/2
  [ADC_IDC] -> Mux/1
  DC Bus Current Measurement Module/1(ADC OUT) -> [ADC_IDC]
  DC Bus Current Measurement Module/2(Scope View (p.u.)) -> Scope13/1
  DC Bus Current Measurement Module/3(Sample & Hold View) -> Scope14/1
  [SampleTrig] -> DC Bus Current Measurement Module/1(Sample Trigger)
  Capactor Voltage Uab Measurement Module1/3(Sample & Hold View) -> Scope8/1
  Capactor Voltage Uab Measurement Module1/2(Scope View (p.u.)) -> Scope9/1
  Capactor Voltage Uab Measurement Module1/1(ADC OUT) -> [ADC_UDC]
  [SampleTrig] -> Capactor Voltage Uab Measurement Module1/1(Sample Trigger)
  Capactor Voltage Ubc Measurement Module5/2(Scope View (p.u.)) -> Scope4/1
  [SampleTrig] -> Capactor Voltage Ubc Measurement Module5/1(Sample Trigger)
  Capactor Voltage Ubc Measurement Module5/3(Sample & Hold View) -> Scope3/1
  Capactor Voltage Ubc Measurement Module5/1(ADC OUT) -> [ADC_UBC2]
  Capactor Voltage Uab Measurement Module/1(ADC OUT) -> [ADC_UAB2]
  Capactor Voltage Uab Measurement Module/3(Sample & Hold View) -> Scope1/1
  Capactor Voltage Uab Measurement Module/2(Scope View (p.u.)) -> Scope2/1
  [SampleTrig] -> Capactor Voltage Uab Measurement Module/1(Sample Trigger)
  [EnableTag] -> Single Phase Full Bridge (Duty Model) phase W/1
  Single Phase Full Bridge (Duty Model) phase W/1 -> Terminator1/1
  Capactor Current Ia Measurement Module/1(ADC OUT) -> [ADC_IA2]
  Capactor Current Ia Measurement Module/3(Sample & Hold View) -> Scope12/1
  [SampleTrig] -> Capactor Current Ia Measurement Module/1(Sample Trigger)
  Capactor Current Ia Measurement Module/2(Scope View (p.u.)) -> Scope11/1
  Capactor Current Ib Measurement Module/1(ADC OUT) -> [ADC_IB2]
  Capactor Current Ib Measurement Module/3(Sample & Hold View) -> Scope10/1
  [SampleTrig] -> Capactor Current Ib Measurement Module/1(Sample Trigger)
  Capactor Current Ib Measurement Module/2(Scope View (p.u.)) -> Scope7/1
  [SampleTrig] -> Capactor Current Ic Measurement Module/1(Sample Trigger)
  Capactor Current Ic Measurement Module/3(Sample & Hold View) -> Scope6/1
  Capactor Current Ic Measurement Module/2(Scope View (p.u.)) -> Scope5/1
  Capactor Current Ic Measurement Module/1(ADC OUT) -> [ADC_IC2]
  Demux/3 -> [BPWM6]
  [BPWM6] -> Single Phase Full Bridge (Duty Model) phase W/2
  [SampleTrig] -> Trig/1
  Mux/1 -> ADC Port/1
  Demux/2 -> [BPWM5]
  Demux/1 -> [BPWM4]
  PWM CMP/1 -> Demux/1
  Enable/1 -> [EnableTag]
  [BPWM5] -> Single Phase Full Bridge (Duty Model) phase V/2(PWM CMP)
  [EnableTag] -> Single Phase Full Bridge (Duty Model) phase V/1(Enable)
  Single Phase Full Bridge (Duty Model) phase V/1(Sample Trigger Output) -> Terminator3/1
  [EnableTag] -> Single Phase Full Bridge (Duty Model) phase U/1(Enable)
  [BPWM4] -> Single Phase Full Bridge (Duty Model) phase U/2(PWM CMP)
  Single Phase Full Bridge (Duty Model) phase U/1(Sample Trigger Output) -> [SampleTrig]
  connections:
  DC Bus Current Measurement Module/LConn2 -- DC_Bus_Current_Sensor/LConn1 -- DC_BUS-/RConn1
  Single Phase Full Bridge (Duty Model) phase V/RConn1 -- Series RLC Branch1/LConn1
  Single Phase Full Bridge (Duty Model) phase W/RConn1 -- Series RLC Branch2/LConn1
  Capactor Current Ia Measurement Module/LConn1 -- Capactor Voltage Uab Measurement Module/LConn1 -- Series RLC Branch4/RConn1 -- Series RLC Branch5/RConn1 -- Series RLC Branch/RConn1 -- Grid_Current_Sensor2/RConn1
  Single Phase Full Bridge (Duty Model) phase U/RConn1 -- Series RLC Branch/LConn1
  Series RLC Branch8/LConn1 -- AC_BUS_N/RConn1 -- Series RLC Branch7/LConn1 -- Series RLC Branch6/LConn1 -- Series RLC Branch4/LConn1 -- Series RLC Branch5/LConn1 -- Series RLC Branch3/LConn1
  Grid_Current_Sensor2/LConn1 -- Capactor Current Ia Measurement Module/LConn2 -- AC_BUS_A/RConn1
  AC_BUS_B/RConn1 -- Capactor Current Ib Measurement Module/LConn2 -- Grid_Current_Sensor1/LConn1
  Capactor Current Ic Measurement Module/LConn2 -- AC_BUS_C/RConn1 -- Grid_Current_Sensor/LConn1
  Series RLC Branch2/RConn1 -- Series RLC Branch7/RConn1 -- Series RLC Branch8/RConn1 -- Capactor Voltage Ubc Measurement Module5/LConn2 -- Grid_Current_Sensor/RConn1 -- Capactor Current Ic Measurement Module/LConn1
  Capactor Current Ib Measurement Module/LConn1 -- Capactor Voltage Uab Measurement Module/LConn2 -- Capactor Voltage Ubc Measurement Module5/LConn1 -- Series RLC Branch1/RConn1 -- Series RLC Branch6/RConn1 -- Series RLC Branch3/RConn1 -- Grid_Current_Sensor1/RConn1
  Capactor Voltage Uab Measurement Module1/LConn1 -- Single Phase Full Bridge (Duty Model) phase V/LConn1 -- Single Phase Full Bridge (Duty Model) phase U/LConn1 -- Single Phase Full Bridge (Duty Model) phase W/LConn1 -- Input_C_EPR/LConn1 -- Input_C/LConn1 -- DC_BUS+/RConn1
  DC Bus Current Measurement Module/LConn1 -- DC_Bus_Current_Sensor/RConn1 -- Single Phase Full Bridge (Duty Model) phase V/RConn2 -- Single Phase Full Bridge (Duty Model) phase U/RConn2 -- Single Phase Full Bridge (Duty Model) phase W/RConn2 -- Input_C_EPR/RConn1 -- Capactor Voltage Uab Measurement Module1/LConn2 -- Input_C/RConn1

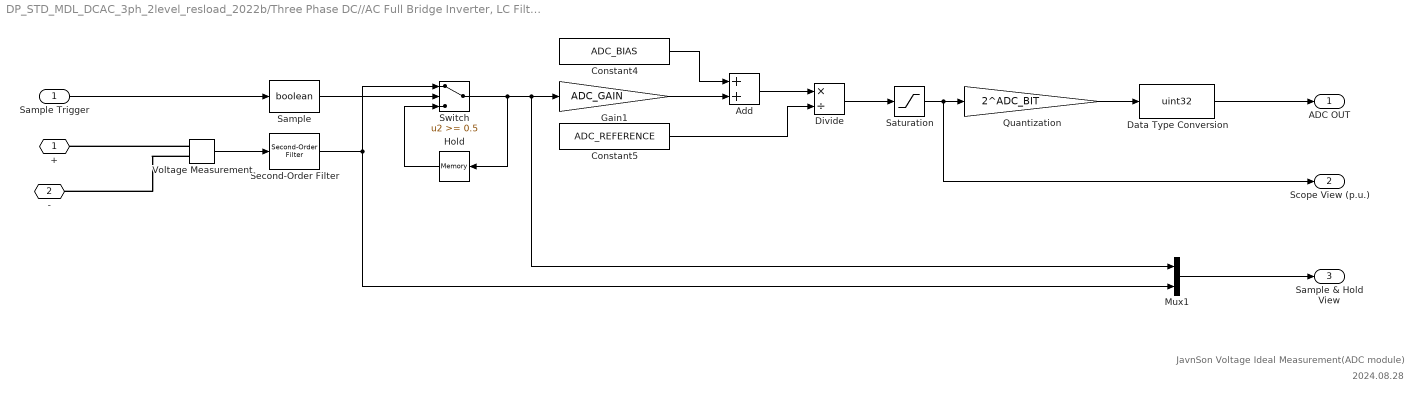
== system DP_STD_MDL_DCAC_3ph_2level_resload_2022b/Three Phase DC//AC Full Bridge Inverter, LC Filter (GMP STD MDL)/Capactor Current Ia Measurement Module ==
  note: JavnSon Voltage Ideal Measurement(ADC module)
  note: 2024.08.28
  Sample Trigger : Inport
  Add : Sum
  Constant4 : Constant  Value=ADC_BIAS
  Constant5 : Constant  Value=ADC_REFERENCE
  Data Type Conversion : DataTypeConversion  OutDataTypeStr=uint32  ConvertRealWorld=Stored Integer (SI)  SaturateOnIntegerOverflow=off  RndMeth=Floor
  Divide : Product  Inputs=*/
  Gain1 : Gain  Gain=ADC_GAIN
  Hold : Memory  InitialCondition=ADC_INIT  LinearizeAsDelay=on
  Mux1 : Mux  Inputs=2
  Quantization : Gain  Gain=2^ADC_BIT
  Sample : DataTypeConversion  OutDataTypeStr=boolean  SaturateOnIntegerOverflow=off  RndMeth=Floor
  Saturation : Saturate  UpperLimit=1  LowerLimit=0
  Second-Order Filter : spsSecondOrderFilterLib/Second-Order Filter  FilterType=Lowpass  Fo=cut_frequency  Zeta=0.707  Ts=0  Initialize=off  Vac_Init="[0,  0,  60]"  Vdc_Init=0  PlotResponse=off  FreqRange=[0, 500, 1]
  Switch : Switch  Threshold=0.5
  Voltage Measurement : spsVoltageMeasurementLib/Voltage Measurement  PhasorSimulation=off  OutputType=Complex  PSBequivalent=0
  + : PMIOPort  Side=Left
  - : PMIOPort  Port=2  Side=Left
  ADC OUT : Outport
  Scope View (p.u.) : Outport  Port=2
  Sample & Hold View : Outport  Port=3
  wires:
  Second-Order Filter/1 -> Mux1/2, Switch/1
  Hold/1 -> Switch/3
  Switch/1 -> Hold/1, Mux1/1, Gain1/1
  Divide/1 -> Saturation/1
  Voltage Measurement/1 -> Second-Order Filter/1
  Saturation/1 -> Scope View (p.u.)/1, Quantization/1
  Constant4/1 -> Add/1
  Gain1/1 -> Add/2
  Sample Trigger/1 -> Sample/1
  Data Type Conversion/1 -> ADC OUT/1
  Mux1/1 -> Sample & Hold View/1
  Quantization/1 -> Data Type Conversion/1
  Constant5/1 -> Divide/2
  Add/1 -> Divide/1
  Sample/1 -> Switch/2
  connections:
  Voltage Measurement/LConn1 -- +/RConn1
  Voltage Measurement/LConn2 -- -/RConn1

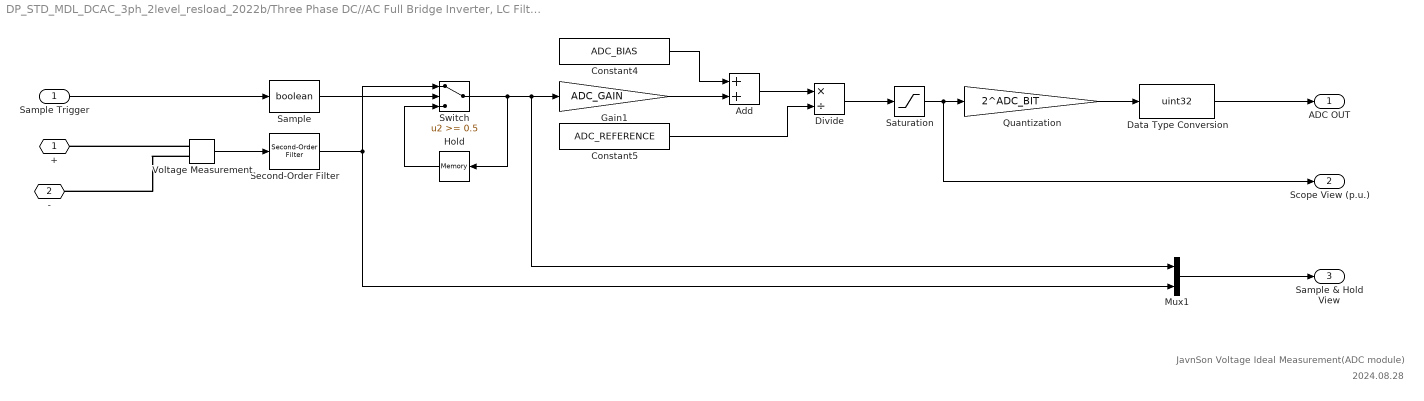
== system DP_STD_MDL_DCAC_3ph_2level_resload_2022b/Three Phase DC//AC Full Bridge Inverter, LC Filter (GMP STD MDL)/Capactor Current Ib Measurement Module ==
  note: JavnSon Voltage Ideal Measurement(ADC module)
  note: 2024.08.28
  Sample Trigger : Inport
  Add : Sum
  Constant4 : Constant  Value=ADC_BIAS
  Constant5 : Constant  Value=ADC_REFERENCE
  Data Type Conversion : DataTypeConversion  OutDataTypeStr=uint32  ConvertRealWorld=Stored Integer (SI)  SaturateOnIntegerOverflow=off  RndMeth=Floor
  Divide : Product  Inputs=*/
  Gain1 : Gain  Gain=ADC_GAIN
  Hold : Memory  InitialCondition=ADC_INIT  LinearizeAsDelay=on
  Mux1 : Mux  Inputs=2
  Quantization : Gain  Gain=2^ADC_BIT
  Sample : DataTypeConversion  OutDataTypeStr=boolean  SaturateOnIntegerOverflow=off  RndMeth=Floor
  Saturation : Saturate  UpperLimit=1  LowerLimit=0
  Second-Order Filter : spsSecondOrderFilterLib/Second-Order Filter  FilterType=Lowpass  Fo=cut_frequency  Zeta=0.707  Ts=0  Initialize=off  Vac_Init="[0,  0,  60]"  Vdc_Init=0  PlotResponse=off  FreqRange=[0, 500, 1]
  Switch : Switch  Threshold=0.5
  Voltage Measurement : spsVoltageMeasurementLib/Voltage Measurement  PhasorSimulation=off  OutputType=Complex  PSBequivalent=0
  + : PMIOPort  Side=Left
  - : PMIOPort  Port=2  Side=Left
  ADC OUT : Outport
  Scope View (p.u.) : Outport  Port=2
  Sample & Hold View : Outport  Port=3
  wires:
  Second-Order Filter/1 -> Mux1/2, Switch/1
  Hold/1 -> Switch/3
  Switch/1 -> Hold/1, Mux1/1, Gain1/1
  Divide/1 -> Saturation/1
  Voltage Measurement/1 -> Second-Order Filter/1
  Saturation/1 -> Scope View (p.u.)/1, Quantization/1
  Constant4/1 -> Add/1
  Gain1/1 -> Add/2
  Sample Trigger/1 -> Sample/1
  Data Type Conversion/1 -> ADC OUT/1
  Mux1/1 -> Sample & Hold View/1
  Quantization/1 -> Data Type Conversion/1
  Constant5/1 -> Divide/2
  Add/1 -> Divide/1
  Sample/1 -> Switch/2
  connections:
  Voltage Measurement/LConn1 -- +/RConn1
  Voltage Measurement/LConn2 -- -/RConn1

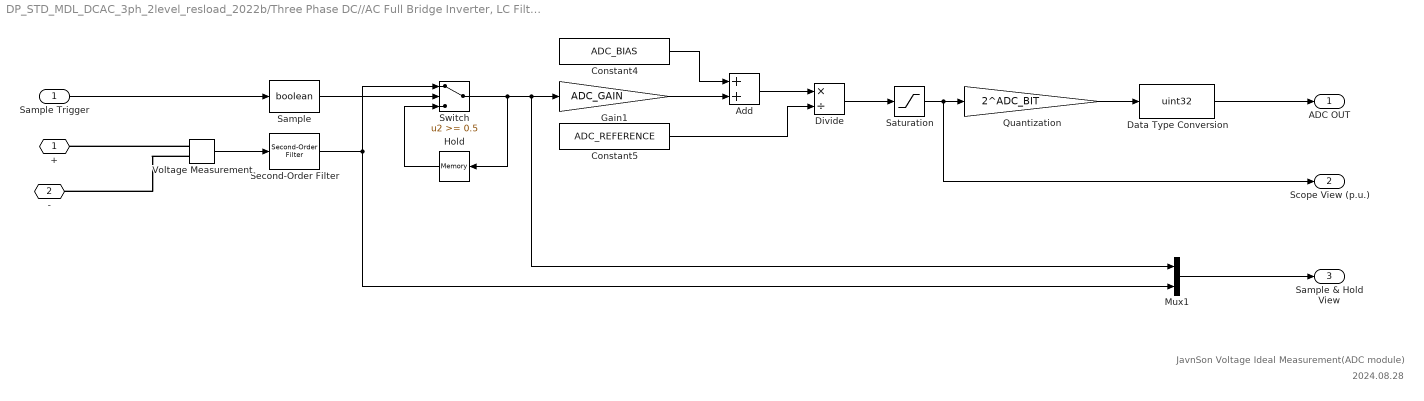
== system DP_STD_MDL_DCAC_3ph_2level_resload_2022b/Three Phase DC//AC Full Bridge Inverter, LC Filter (GMP STD MDL)/Capactor Current Ic Measurement Module ==
  note: JavnSon Voltage Ideal Measurement(ADC module)
  note: 2024.08.28
  Sample Trigger : Inport
  Add : Sum
  Constant4 : Constant  Value=ADC_BIAS
  Constant5 : Constant  Value=ADC_REFERENCE
  Data Type Conversion : DataTypeConversion  OutDataTypeStr=uint32  ConvertRealWorld=Stored Integer (SI)  SaturateOnIntegerOverflow=off  RndMeth=Floor
  Divide : Product  Inputs=*/
  Gain1 : Gain  Gain=ADC_GAIN
  Hold : Memory  InitialCondition=ADC_INIT  LinearizeAsDelay=on
  Mux1 : Mux  Inputs=2
  Quantization : Gain  Gain=2^ADC_BIT
  Sample : DataTypeConversion  OutDataTypeStr=boolean  SaturateOnIntegerOverflow=off  RndMeth=Floor
  Saturation : Saturate  UpperLimit=1  LowerLimit=0
  Second-Order Filter : spsSecondOrderFilterLib/Second-Order Filter  FilterType=Lowpass  Fo=cut_frequency  Zeta=0.707  Ts=0  Initialize=off  Vac_Init="[0,  0,  60]"  Vdc_Init=0  PlotResponse=off  FreqRange=[0, 500, 1]
  Switch : Switch  Threshold=0.5
  Voltage Measurement : spsVoltageMeasurementLib/Voltage Measurement  PhasorSimulation=off  OutputType=Complex  PSBequivalent=0
  + : PMIOPort  Side=Left
  - : PMIOPort  Port=2  Side=Left
  ADC OUT : Outport
  Scope View (p.u.) : Outport  Port=2
  Sample & Hold View : Outport  Port=3
  wires:
  Second-Order Filter/1 -> Mux1/2, Switch/1
  Hold/1 -> Switch/3
  Switch/1 -> Hold/1, Mux1/1, Gain1/1
  Divide/1 -> Saturation/1
  Voltage Measurement/1 -> Second-Order Filter/1
  Saturation/1 -> Scope View (p.u.)/1, Quantization/1
  Constant4/1 -> Add/1
  Gain1/1 -> Add/2
  Sample Trigger/1 -> Sample/1
  Data Type Conversion/1 -> ADC OUT/1
  Mux1/1 -> Sample & Hold View/1
  Quantization/1 -> Data Type Conversion/1
  Constant5/1 -> Divide/2
  Add/1 -> Divide/1
  Sample/1 -> Switch/2
  connections:
  Voltage Measurement/LConn1 -- +/RConn1
  Voltage Measurement/LConn2 -- -/RConn1

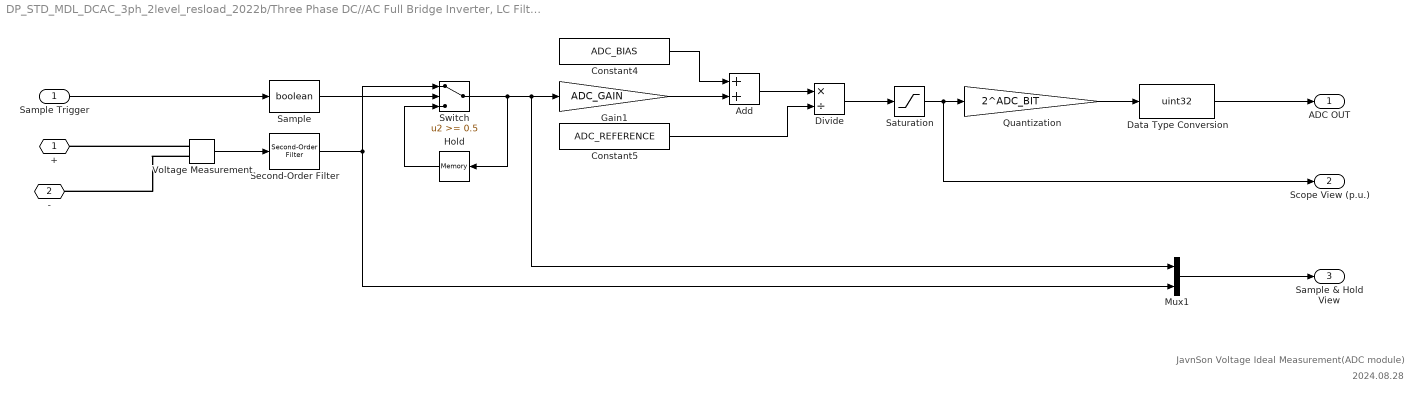
== system DP_STD_MDL_DCAC_3ph_2level_resload_2022b/Three Phase DC//AC Full Bridge Inverter, LC Filter (GMP STD MDL)/Capactor Voltage Uab Measurement Module ==
  note: 2024.08.28
  note: JavnSon Voltage Ideal Measurement(ADC module)
  Sample Trigger : Inport
  Add : Sum
  Constant4 : Constant  Value=ADC_BIAS
  Constant5 : Constant  Value=ADC_REFERENCE
  Data Type Conversion : DataTypeConversion  OutDataTypeStr=uint32  ConvertRealWorld=Stored Integer (SI)  SaturateOnIntegerOverflow=off  RndMeth=Floor
  Divide : Product  Inputs=*/
  Gain1 : Gain  Gain=ADC_GAIN
  Hold : Memory  InitialCondition=ADC_INIT  LinearizeAsDelay=on
  Mux1 : Mux  Inputs=2
  Quantization : Gain  Gain=2^ADC_BIT
  Sample : DataTypeConversion  OutDataTypeStr=boolean  SaturateOnIntegerOverflow=off  RndMeth=Floor
  Saturation : Saturate  UpperLimit=1  LowerLimit=0
  Second-Order Filter : spsSecondOrderFilterLib/Second-Order Filter  FilterType=Lowpass  Fo=cut_frequency  Zeta=0.707  Ts=0  Initialize=off  Vac_Init="[0,  0,  60]"  Vdc_Init=0  PlotResponse=off  FreqRange=[0, 500, 1]
  Switch : Switch  Threshold=0.5
  Voltage Measurement : spsVoltageMeasurementLib/Voltage Measurement  PhasorSimulation=off  OutputType=Complex  PSBequivalent=0
  + : PMIOPort  Side=Left
  - : PMIOPort  Port=2  Side=Left
  ADC OUT : Outport
  Scope View (p.u.) : Outport  Port=2
  Sample & Hold View : Outport  Port=3
  wires:
  Sample/1 -> Switch/2
  Add/1 -> Divide/1
  Constant5/1 -> Divide/2
  Quantization/1 -> Data Type Conversion/1
  Mux1/1 -> Sample & Hold View/1
  Data Type Conversion/1 -> ADC OUT/1
  Sample Trigger/1 -> Sample/1
  Gain1/1 -> Add/2
  Constant4/1 -> Add/1
  Saturation/1 -> Quantization/1, Scope View (p.u.)/1
  Voltage Measurement/1 -> Second-Order Filter/1
  Divide/1 -> Saturation/1
  Switch/1 -> Gain1/1, Mux1/1, Hold/1
  Hold/1 -> Switch/3
  Second-Order Filter/1 -> Switch/1, Mux1/2
  connections:
  Voltage Measurement/LConn2 -- -/RConn1
  Voltage Measurement/LConn1 -- +/RConn1
